simulink model "XY_1_pen_sim"  (R2024b)
settings: Solver=ode4  StartTime=0.0  StopTime=T_run  FixedStep=Ts_plant  RelTol=1e-3
StopFcn:
  | XY_stop
values from neighbouring files (symbols this model uses):
  alpha_s = 0    [XY_setup.m]
  anim_Ts = 0.2    [XY_setup.m]
  animate = 1    [XY_1_pen_sim_run.m]    (also in XY_compare.m = 0; XY_run_all.m; XY_setup.m)
  B_eff = 0.30    (= 0.3)    [XY_setup.m]
  b_trk = 0.28    [XY_setup.m]
  d_reach = 0.03    [XY_setup.m]
  db_v = 47    [XY_setup.m]
  db_w = 20    [XY_setup.m]
  dist_p = [slip_k; wob_amp; wob_f]    [XY_setup.m]
  dyn_p = [m_r; l_trk; b_trk; mu_l; mu_t; N_mag; g_acc]    [XY_setup.m]
  F_max = 200    [XY_setup.m]
  imu_drift = deg2rad(0.02)    [XY_setup.m]
  imu_sigma = deg2rad(0.3)    [XY_setup.m]
  imu_Ts = 0.01    [XY_setup.m]
  K_c = 0    [XY_setup.m]
  K_ci = 0    [XY_setup.m]
  K_dist = 1.0    (= 1)    [XY_setup.m]
  K_ptheta = 1.4    [XY_setup.m]
  k_pwm = v_full/(400 - pwm_dz)    (= 0.000540540540541)    [XY_setup.m]
  K_px = 0.3    [XY_setup.m]
  K_py = 5.0    (= 5)    [XY_setup.m]
  K_yaw = 2.0    (= 2)    [XY_setup.m]
  Ki_v = 15000    [XY_setup.m]
  Ki_w = 15000    [XY_setup.m]
  Kp_v = 1500    [XY_setup.m]
  Kp_w = 1500    [XY_setup.m]
  L_r = sqrt((l_trk^2 + b_trk^2)/12)    [XY_setup.m]
  line_post = 0.04    [XY_setup.m]
  line_pre = 0.06    [XY_setup.m]
  pen_A = [-0.70; 0.30]    [XY_setup.m]
  pen_B = [ 0.50; 0.30]    [XY_setup.m]
  pen_d = r_pen0 - r_tag    [XY_setup.m]
  psi0 = pi/2    (= 1.57079632679)    [XY_setup.m]
  pwm_dz = 30    [XY_setup.m]
  q0 = [-0.85; 0.10; pi/2]    [XY_setup.m]
  q0c = [q0(1:2) - [cos(q0(3)) -sin(q0(3)); sin(q0(3)) cos(q0(3))] * r_tag; q0(3)]    [XY_setup.m]
  r_tag = [-0.080;  0.060]    [XY_setup.m]
  stage_acc = 500    [XY_setup.m]
  stage_c = stage_travel/2    (= 50.8)    [XY_setup.m]
  stage_cmd_Ts = 0.04    [XY_setup.m]
  stage_delay = 0.01    [XY_setup.m]
  stage_Fv_F = [32 32 29 26.5 25 22  20 17.5 14  9]    [XY_setup.m]
  stage_Fv_v = [0  2  7  13  20  32  45  60  80  104]    [XY_setup.m]
  stage_travel = 101.6    [XY_setup.m]
  stage_Ts = 0.05    [XY_setup.m]
  stage_vcmd = 0.8*stage_vmax    (= 83.2)    [XY_setup.m]
  stage_vmax = 104    [XY_setup.m]
  stg_p = [m_sx; m_sy; c_s; Kp_s; Kd_s; Ki_s; g_acc]    [XY_compare.m]    (also in XY_setup.m)
  tau_pred = 0    [XY_setup.m]
  th_tol = deg2rad(1)    [XY_setup.m]
  trk_A = -eye(2)/tau_trk    [XY_setup.m]
  trk_B = eye(2)/tau_trk    [XY_setup.m]
  trk_C = eye(2)    [XY_setup.m]
  trk_D = zeros(2)    [XY_setup.m]
  Ts_ctrl = 0.01    [XY_setup.m]
  v_full = 0.20    (= 0.2)    [XY_setup.m]
  v_max = 0.20    (= 0.2)    [XY_setup.m]
  v_ref = 0.03    [XY_setup.m]
  w_full = 2*k_pwm*(400 - db_w)/B_eff    (= 1.36936936937)    [XY_setup.m]
  w_max = deg2rad(45)    [XY_setup.m]
  x = c(1) + s(1)/2*[-1 1 1 -1 -1 1 1 -1]    [XY_animate.m]
  x_s0 = [stage_c; stage_c; 0; 0; 0; 0] .* [1e-3; 1e-3; 1; 1; 1; 1]    [XY_setup.m]
  x_t0 = [stage_c; stage_c; 0; 0]    [XY_setup.m]
  y = c(2) + s(2)/2*[-1 -1 1 1 -1 -1 1 1]    [XY_animate.m]    (also in build_xy_models.m = q(2))
  zk_delay = 0.05    [XY_setup.m]
  zk_sigma = 0.0010    (= 0.001)    [XY_setup.m]
  zk_Ts = 0.05    [XY_setup.m]
  zk_xsign = -1    [XY_setup.m]
  zk_ywall = 0.02    [XY_setup.m]
undefined symbols (not defined in the file or in its folder): orientation, point, quaternion, twist
libraries: ros2lib x20, simulink x4, slpidlib x2
(part 1 of 2)
settings Model: PacingRate=4  Creator=admin  LastModifiedBy=admin
settings DataIOCC: ReturnWorkspaceOutputs=off

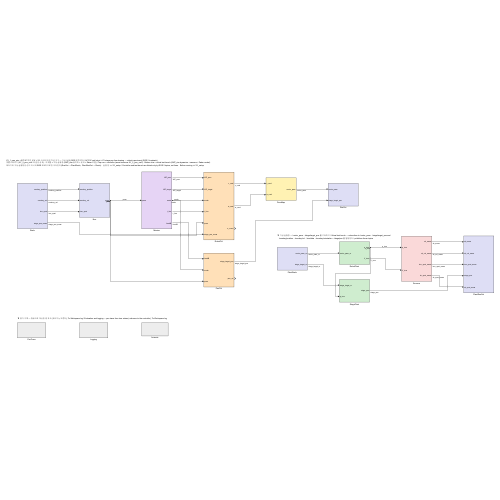
[thumbnail: Simulink's stored preview of the top-level diagram]
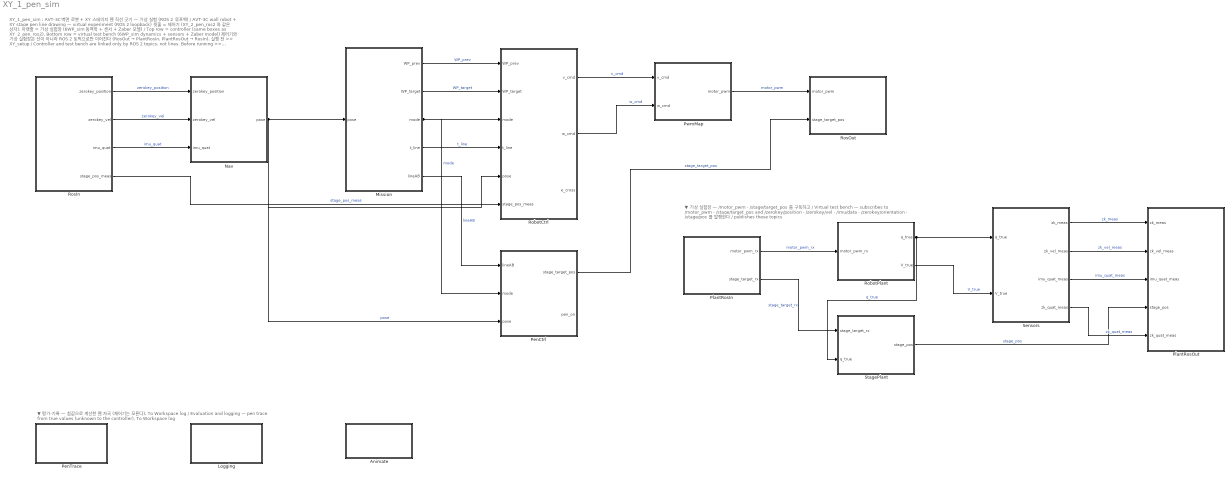
== system XY_1_pen_sim ==
  note: XY_1_pen_sim : AVT-3C 벽면 로봇 + XY 스테이지 펜 직선 긋기 — 가상 실험 (ROS 2 루프백) / AVT-3C wall robot + XY stage pen line drawing — virtual experiment (ROS 2 loopback)
      | 윗줄 = 제어기 (XY_2_pen_ros2 와 같은 상자).  아랫줄 = 가상 실험장 (6WP_sim 동역학 + 센서 + Zaber 모델) / Top row = controller (same boxes as XY_2_pen_ros2).  Bottom row = virtual test bench (6WP_sim dynamics + sensors + Zaber model)
      | 제어기와 가상 실험장은 선이 아니라 ROS 2 토픽으로만 이어진다 (RosOut → PlantRosIn,  PlantRosOut → RosIn).   실행 전 >> XY_setup / Controller and test bench are linked only by ROS 2 topics, not lines.   Before running >> XY_setup
  note: ▼ 가상 실험장 — /motor_pwm · /stage/target_pos 를 구독하고 / Virtual test bench — subscribes to /motor_pwm · /stage/target_pos and
      |    /zerokey/position · /zerokey/vel · /imu/data · /zerokey/orientation · /stage/pos 를 발행한다 / publishes these topics
  note: ▼ 평가·기록 — 참값으로 계산한 펜 자국 (제어기는 모른다), To Workspace log / Evaluation and logging — pen trace from true values (unknown to the controller), To Workspace log
  Animate : Subsystem
  Logging : Subsystem
  Mission : Subsystem
  Nav : Subsystem
  PenCtrl : Subsystem
  PenTrace : Subsystem
  PlantRosIn : Subsystem
  PlantRosOut : Subsystem
  PwmMap : Subsystem
  RobotCtrl : Subsystem
  RobotPlant : Subsystem
  RosIn : Subsystem
  RosOut : Subsystem
  Sensors : Subsystem
  StagePlant : Subsystem
  wires:
  Nav/1(pose) -> Mission/1(pose), PenCtrl/3(pose), RobotCtrl/5(pose)  "pose"
  RosIn/1(zerokey_position) -> Nav/1(zerokey_position)  "zerokey_position"
  RosIn/2(zerokey_vel) -> Nav/2(zerokey_vel)  "zerokey_vel"
  RosIn/3(imu_quat) -> Nav/3(imu_quat)  "imu_quat"
  Mission/5(lineAB) -> PenCtrl/1(lineAB)  "lineAB"
  Mission/3(mode) -> PenCtrl/2(mode), RobotCtrl/3(mode)  "mode"
  Sensors/1(zk_meas) -> PlantRosOut/1(zk_meas)  "zk_meas"
  Sensors/2(zk_vel_meas) -> PlantRosOut/2(zk_vel_meas)  "zk_vel_meas"
  Sensors/3(imu_quat_meas) -> PlantRosOut/3(imu_quat_meas)  "imu_quat_meas"
  StagePlant/1(stage_pos) -> PlantRosOut/4(stage_pos)  "stage_pos"
  Sensors/4(zk_quat_meas) -> PlantRosOut/5(zk_quat_meas)  "zk_quat_meas"
  RobotCtrl/1(v_cmd) -> PwmMap/1(v_cmd)  "v_cmd"
  RobotCtrl/2(w_cmd) -> PwmMap/2(w_cmd)  "w_cmd"
  Mission/1(WP_prev) -> RobotCtrl/1(WP_prev)  "WP_prev"
  Mission/2(WP_target) -> RobotCtrl/2(WP_target)  "WP_target"
  Mission/4(t_line) -> RobotCtrl/4(t_line)  "t_line"
  RosIn/4(stage_pos_meas) -> RobotCtrl/6(stage_pos_meas)  "stage_pos_meas"
  PlantRosIn/1(motor_pwm_rx) -> RobotPlant/1(motor_pwm_rx)  "motor_pwm_rx"
  PwmMap/1(motor_pwm) -> RosOut/1(motor_pwm)  "motor_pwm"
  PenCtrl/1(stage_target_pos) -> RosOut/2(stage_target_pos)  "stage_target_pos"
  RobotPlant/1(q_true) -> Sensors/1(q_true), StagePlant/2(q_true)  "q_true"
  RobotPlant/2(V_true) -> Sensors/2(V_true)  "V_true"
  PlantRosIn/2(stage_target_rx) -> StagePlant/1(stage_target_rx)  "stage_target_rx"

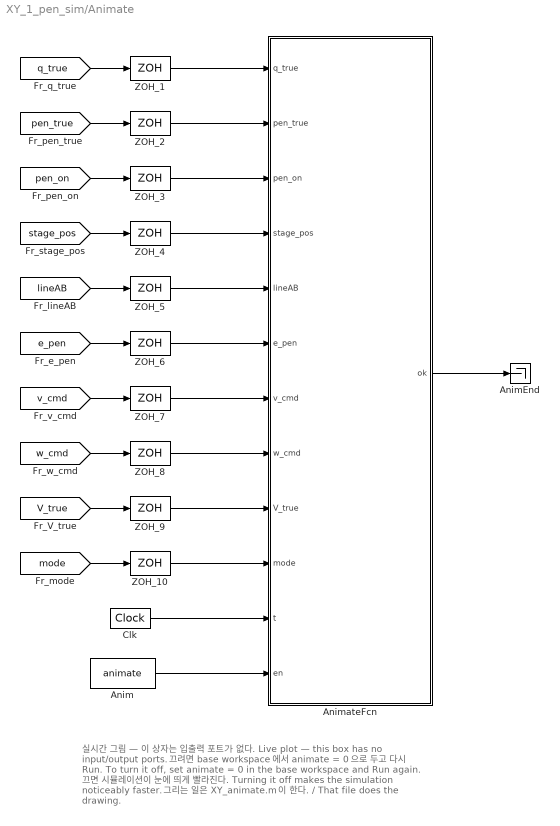
== system XY_1_pen_sim/Animate ==
  note: 실시간 그림 — 이 상자는 입출력 포트가 없다.
      | Live plot — this box has no input/output ports.
      | 끄려면 base workspace 에서  animate = 0  으로 두고 다시 Run.
      | To turn it off, set  animate = 0  in the base workspace and Run again.
      | 끄면 시뮬레이션이 눈에 띄게 빨라진다.
      | Turning it off makes the simulation noticeably faster.
      | 그리는 일은 XY_animate.m 이 한다. / That file does the drawing.
  Anim : Constant  Value=animate
  AnimEnd : Terminator
  AnimateFcn : MATLAB Function  TreatAsAtomicUnit=on
  Clk : DigitalClock  SampleTime=anim_Ts
  ZOH_{1..10} (10 alike) : ZeroOrderHold  SampleTime=anim_Ts
  wires:
  Clk/1 -> AnimateFcn/11(t)
  Anim/1 -> AnimateFcn/12(en)
  AnimateFcn/1(ok) -> AnimEnd/1
  [q_true] -> ZOH_1/1
  ZOH_1/1 -> AnimateFcn/1(q_true)
  [pen_true] -> ZOH_2/1
  ZOH_2/1 -> AnimateFcn/2(pen_true)
  [pen_on] -> ZOH_3/1
  ZOH_3/1 -> AnimateFcn/3(pen_on)
  [stage_pos] -> ZOH_4/1
  ZOH_4/1 -> AnimateFcn/4(stage_pos)
  [lineAB] -> ZOH_5/1
  ZOH_5/1 -> AnimateFcn/5(lineAB)
  [e_pen] -> ZOH_6/1
  ZOH_6/1 -> AnimateFcn/6(e_pen)
  [v_cmd] -> ZOH_7/1
  ZOH_7/1 -> AnimateFcn/7(v_cmd)
  [w_cmd] -> ZOH_8/1
  ZOH_8/1 -> AnimateFcn/8(w_cmd)
  [V_true] -> ZOH_9/1
  ZOH_9/1 -> AnimateFcn/9(V_true)
  [mode] -> ZOH_10/1
  ZOH_10/1 -> AnimateFcn/10(mode)

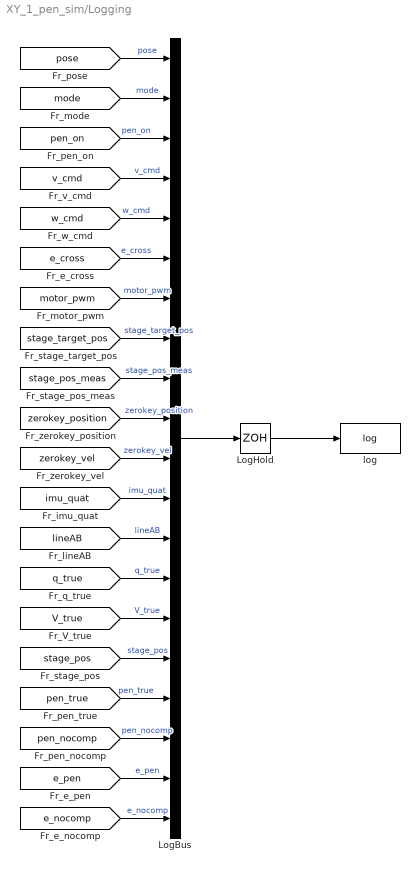
== system XY_1_pen_sim/Logging ==
  LogBus : BusCreator  Inputs=20
  LogHold : ZeroOrderHold  Description=이산: 기록 주기 (제어기 주기와 같다) / Discrete: logging period (same as the controller period)  SampleTime=Ts_ctrl
  log : ToWorkspace  VariableName=log  SaveFormat=Timeseries  SampleTime=Ts_ctrl
  wires:
  [pose] -> LogBus/1  "pose"
  [mode] -> LogBus/2  "mode"
  [pen_on] -> LogBus/3  "pen_on"
  [v_cmd] -> LogBus/4  "v_cmd"
  [w_cmd] -> LogBus/5  "w_cmd"
  [e_cross] -> LogBus/6  "e_cross"
  [motor_pwm] -> LogBus/7  "motor_pwm"
  [stage_target_pos] -> LogBus/8  "stage_target_pos"
  [stage_pos_meas] -> LogBus/9  "stage_pos_meas"
  [zerokey_position] -> LogBus/10  "zerokey_position"
  [zerokey_vel] -> LogBus/11  "zerokey_vel"
  [imu_quat] -> LogBus/12  "imu_quat"
  [lineAB] -> LogBus/13  "lineAB"
  [q_true] -> LogBus/14  "q_true"
  [V_true] -> LogBus/15  "V_true"
  [stage_pos] -> LogBus/16  "stage_pos"
  [pen_true] -> LogBus/17  "pen_true"
  [pen_nocomp] -> LogBus/18  "pen_nocomp"
  [e_pen] -> LogBus/19  "e_pen"
  [e_nocomp] -> LogBus/20  "e_nocomp"
  LogBus/1 -> LogHold/1
  LogHold/1 -> log/1

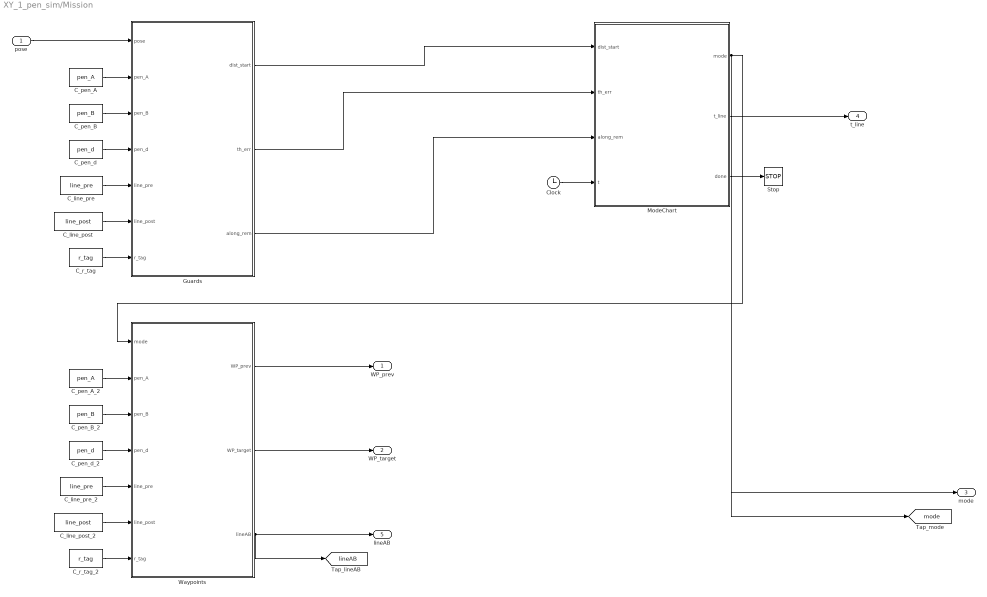
== system XY_1_pen_sim/Mission ==
  pose : Inport
  C_line_post : Constant  Value=line_post
  C_line_post_2 : Constant  Value=line_post
  C_line_pre : Constant  Value=line_pre
  C_line_pre_2 : Constant  Value=line_pre
  C_pen_A : Constant  Value=pen_A
  C_pen_A_2 : Constant  Value=pen_A
  C_pen_B : Constant  Value=pen_B
  C_pen_B_2 : Constant  Value=pen_B
  C_pen_d : Constant  Value=pen_d
  C_pen_d_2 : Constant  Value=pen_d
  C_r_tag : Constant  Value=r_tag
  C_r_tag_2 : Constant  Value=r_tag
  Clock : Clock
  Guards : MATLAB Function  TreatAsAtomicUnit=on
  ModeChart : Stateflow chart  Description=이산: 모드는 사건 상태 (6WP_sim Chart 와 같은 역할). 전이: 거리 < d_reach, 1 s 뒤 각 오차 < th_tol, 남은 거리 < d_reach, 정지 2 s / Discrete: the mode is an event state (same role as the 6WP_sim Chart). Transitions: distance < d_reach, angle error < th_tol after 1 s, remaining distance < d_reach, stop 2 s  TreatAsAtomicUnit=on
  Stop : Stop
  Waypoints : MATLAB Function  TreatAsAtomicUnit=on
  WP_prev : Outport
  WP_target : Outport  Port=2
  mode : Outport  Port=3
  t_line : Outport  Port=4
  lineAB : Outport  Port=5
  tag scope: lineAB=global, mode=global
  wires:
  pose/1 -> Guards/1(pose)
  C_pen_A/1 -> Guards/2(pen_A)
  C_pen_B/1 -> Guards/3(pen_B)
  C_pen_d/1 -> Guards/4(pen_d)
  C_line_pre/1 -> Guards/5(line_pre)
  C_line_post/1 -> Guards/6(line_post)
  C_r_tag/1 -> Guards/7(r_tag)
  Clock/1 -> ModeChart/4(t)
  ModeChart/2(t_line) -> t_line/1
  ModeChart/3(done) -> Stop/1
  C_pen_A_2/1 -> Waypoints/2(pen_A)
  C_pen_B_2/1 -> Waypoints/3(pen_B)
  C_pen_d_2/1 -> Waypoints/4(pen_d)
  C_line_pre_2/1 -> Waypoints/5(line_pre)
  C_line_post_2/1 -> Waypoints/6(line_post)
  C_r_tag_2/1 -> Waypoints/7(r_tag)
  Waypoints/1(WP_prev) -> WP_prev/1
  Waypoints/2(WP_target) -> WP_target/1
  Waypoints/3(lineAB) -> lineAB/1, [lineAB]
  Guards/3(along_rem) -> ModeChart/3(along_rem)
  Guards/1(dist_start) -> ModeChart/1(dist_start)
  ModeChart/1(mode) -> Waypoints/1(mode), mode/1, [mode]
  Guards/2(th_err) -> ModeChart/2(th_err)

== system XY_1_pen_sim/Nav ==
  zerokey_position : Inport
  zerokey_vel : Inport  Port=2
  imu_quat : Inport  Port=3
  C_psi0 : Constant  Value=psi0
  C_tau_pred : Constant  Value=tau_pred
  C_zk_xsign : Constant  Value=zk_xsign
  NavFcn : MATLAB Function  Description=이산: persistent (첫 요각 기억) — 구독 주기와 같다 / Discrete: persistent (stores the first yaw) — same as the subscription period  TreatAsAtomicUnit=on
  pose : Outport
  tag scope: pose=global
  wires:
  zerokey_position/1 -> NavFcn/1(zerokey_position)
  zerokey_vel/1 -> NavFcn/2(zerokey_vel)
  imu_quat/1 -> NavFcn/3(imu_quat)
  C_psi0/1 -> NavFcn/4(psi0)
  C_tau_pred/1 -> NavFcn/5(tau_pred)
  C_zk_xsign/1 -> NavFcn/6(zk_xsign)
  NavFcn/1(pose) -> pose/1, [pose]

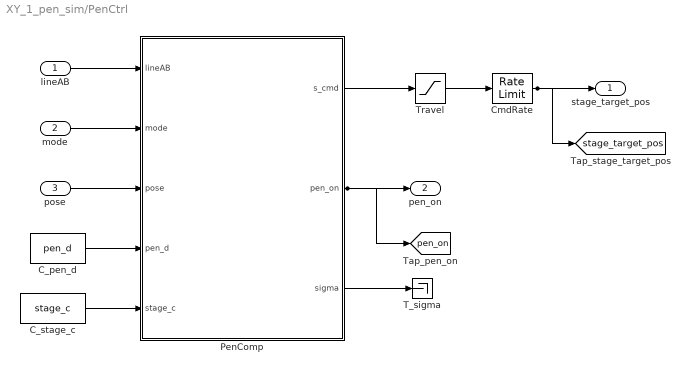
== system XY_1_pen_sim/PenCtrl ==
  lineAB : Inport
  mode : Inport  Port=2
  pose : Inport  Port=3
  C_pen_d : Constant  Value=pen_d
  C_stage_c : Constant  Value=stage_c
  CmdRate : RateLimiter  RisingSlewLimit=stage_vcmd  FallingSlewLimit=-stage_vcmd  SampleTimeMode=inherited  InitialCondition=stage_c
  PenComp : MATLAB Function  TreatAsAtomicUnit=on
  T_sigma : Terminator
  Travel : Saturate  UpperLimit=stage_travel  LowerLimit=0
  stage_target_pos : Outport
  pen_on : Outport  Port=2
  tag scope: pen_on=global, stage_target_pos=global
  wires:
  pose/1 -> PenComp/3(pose)
  lineAB/1 -> PenComp/1(lineAB)
  PenComp/1(s_cmd) -> Travel/1
  C_stage_c/1 -> PenComp/5(stage_c)
  C_pen_d/1 -> PenComp/4(pen_d)
  mode/1 -> PenComp/2(mode)
  PenComp/2(pen_on) -> pen_on/1, [pen_on]
  PenComp/3(sigma) -> T_sigma/1
  Travel/1 -> CmdRate/1
  CmdRate/1 -> stage_target_pos/1, [stage_target_pos]

== system XY_1_pen_sim/PenTrace ==
  C_pen_d : Constant  Value=pen_d
  C_stage_c : Constant  Value=stage_c
  PenTraceFcn : MATLAB Function  TreatAsAtomicUnit=on
  tag scope: e_nocomp=global, e_pen=global, pen_nocomp=global, pen_true=global
  wires:
  [q_true] -> PenTraceFcn/1(q_true)
  [stage_pos] -> PenTraceFcn/2(stage_pos)
  [lineAB] -> PenTraceFcn/3(lineAB)
  C_pen_d/1 -> PenTraceFcn/4(pen_d)
  C_stage_c/1 -> PenTraceFcn/5(stage_c)
  PenTraceFcn/1(pen_true) -> [pen_true]
  PenTraceFcn/2(pen_nocomp) -> [pen_nocomp]
  PenTraceFcn/3(e_pen) -> [e_pen]
  PenTraceFcn/4(e_nocomp) -> [e_nocomp]

== system XY_1_pen_sim/PlantRosIn ==
  IsNew_SubPwm : Terminator
  IsNew_SubStg : Terminator
  Mux_SubPwm : Mux  Inputs=2
  Mux_SubStg : Mux  Inputs=2
  Sel_SubPwm : BusSelector  OutputSignals=x,y
  Sel_SubStg : BusSelector  OutputSignals=x,y
  SubPwm : ros2lib/Subscribe  Description=이산: ROS Subscribe 는 구독 주기로만 돈다 / Discrete: ROS Subscribe runs only at the subscription period  topicSource=Specify your own  topic=/motor_pwm  messageType=geometry_msgs/Point  sampleTime=Ts_ctrl  QOSHistory=Keep last  QOSDepth=1  QOSReliability=Reliable  QOSDurability=Volatile  QOSDeadline=Inf  QOSLifespan=Inf  QOSLiveliness=Automatic  QOSLeaseDuration=Inf  QOSAvoidROSNamespaceConventions=off
  SubStg : ros2lib/Subscribe  Description=이산: ROS Subscribe 는 구독 주기로만 돈다 / Discrete: ROS Subscribe runs only at the subscription period  topicSource=Specify your own  topic=/stage/target_pos  messageType=geometry_msgs/Point  sampleTime=Ts_ctrl  QOSHistory=Keep last  QOSDepth=1  QOSReliability=Reliable  QOSDurability=Volatile  QOSDeadline=Inf  QOSLifespan=Inf  QOSLiveliness=Automatic  QOSLeaseDuration=Inf  QOSAvoidROSNamespaceConventions=off
  motor_pwm_rx : Outport
  stage_target_rx : Outport  Port=2
  wires:
  SubPwm/2 -> Sel_SubPwm/1
  SubPwm/1 -> IsNew_SubPwm/1
  Sel_SubPwm/1 -> Mux_SubPwm/1  "<x>"
  Sel_SubPwm/2 -> Mux_SubPwm/2  "<y>"
  Mux_SubPwm/1 -> motor_pwm_rx/1
  SubStg/2 -> Sel_SubStg/1
  SubStg/1 -> IsNew_SubStg/1
  Sel_SubStg/1 -> Mux_SubStg/1  "<x>"
  Sel_SubStg/2 -> Mux_SubStg/2  "<y>"
  Mux_SubStg/1 -> stage_target_rx/1

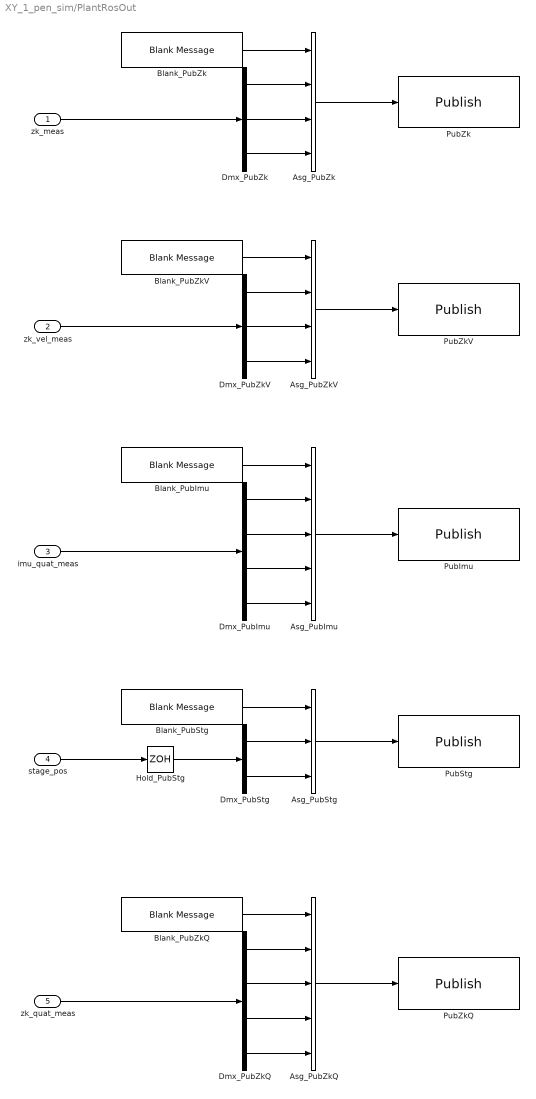
== system XY_1_pen_sim/PlantRosOut ==
  zk_meas : Inport
  zk_vel_meas : Inport  Port=2
  imu_quat_meas : Inport  Port=3
  stage_pos : Inport  Port=4
  zk_quat_meas : Inport  Port=5
  Asg_PubImu : BusAssignment  AssignedSignals=orientation.w,orientation.x,orientation.y,orientation.z
  Asg_PubStg : BusAssignment  AssignedSignals=point.x,point.y
  Asg_PubZk : BusAssignment  AssignedSignals=point.x,point.y,point.z
  Asg_PubZkQ : BusAssignment  AssignedSignals=quaternion.w,quaternion.x,quaternion.y,quaternion.z
  Asg_PubZkV : BusAssignment  AssignedSignals=twist.linear.x,twist.linear.y,twist.linear.z
  Blank_PubImu : ros2lib/Blank Message  messageClass=Message  entityType=sensor_msgs/Imu  messageType=sensor_msgs/Imu  SampleTime=inf
  Blank_PubStg : ros2lib/Blank Message  messageClass=Message  entityType=geometry_msgs/PointStamped  messageType=geometry_msgs/PointStamped  SampleTime=inf
  Blank_PubZk : ros2lib/Blank Message  messageClass=Message  entityType=geometry_msgs/PointStamped  messageType=geometry_msgs/PointStamped  SampleTime=inf
  Blank_PubZkQ : ros2lib/Blank Message  messageClass=Message  entityType=geometry_msgs/QuaternionStamped  messageType=geometry_msgs/QuaternionStamped  SampleTime=inf
  Blank_PubZkV : ros2lib/Blank Message  messageClass=Message  entityType=geometry_msgs/TwistStamped  messageType=geometry_msgs/TwistStamped  SampleTime=inf
  Dmx_PubImu : Demux
  Dmx_PubStg : Demux  Outputs=2
  Dmx_PubZk : Demux  Outputs=3
  Dmx_PubZkQ : Demux
  Dmx_PubZkV : Demux  Outputs=3
  Hold_PubStg : ZeroOrderHold  Description=이산: 발행 주기 / Discrete: publish period  SampleTime=stage_Ts
  PubImu : ros2lib/Publish  topicSource=Specify your own  topic=/imu/data  messageType=sensor_msgs/Imu  QOSHistory=Keep last  QOSDepth=1  QOSReliability=Reliable  QOSDurability=Volatile  QOSDeadline=Inf  QOSLifespan=Inf  QOSLiveliness=Automatic  QOSLeaseDuration=Inf  QOSAvoidROSNamespaceConventions=off
  PubStg : ros2lib/Publish  topicSource=Specify your own  topic=/stage/pos  messageType=geometry_msgs/PointStamped  QOSHistory=Keep last  QOSDepth=1  QOSReliability=Reliable  QOSDurability=Volatile  QOSDeadline=Inf  QOSLifespan=Inf  QOSLiveliness=Automatic  QOSLeaseDuration=Inf  QOSAvoidROSNamespaceConventions=off
  PubZk : ros2lib/Publish  topicSource=Specify your own  topic=/zerokey/position  messageType=geometry_msgs/PointStamped  QOSHistory=Keep last  QOSDepth=1  QOSReliability=Reliable  QOSDurability=Volatile  QOSDeadline=Inf  QOSLifespan=Inf  QOSLiveliness=Automatic  QOSLeaseDuration=Inf  QOSAvoidROSNamespaceConventions=off
  PubZkQ : ros2lib/Publish  topicSource=Specify your own  topic=/zerokey/orientation  messageType=geometry_msgs/QuaternionStamped  QOSHistory=Keep last  QOSDepth=1  QOSReliability=Reliable  QOSDurability=Volatile  QOSDeadline=Inf  QOSLifespan=Inf  QOSLiveliness=Automatic  QOSLeaseDuration=Inf  QOSAvoidROSNamespaceConventions=off
  PubZkV : ros2lib/Publish  topicSource=Specify your own  topic=/zerokey/vel  messageType=geometry_msgs/TwistStamped  QOSHistory=Keep last  QOSDepth=1  QOSReliability=Reliable  QOSDurability=Volatile  QOSDeadline=Inf  QOSLifespan=Inf  QOSLiveliness=Automatic  QOSLeaseDuration=Inf  QOSAvoidROSNamespaceConventions=off
  wires:
  Blank_PubZk/1 -> Asg_PubZk/1
  Dmx_PubZk/1 -> Asg_PubZk/2
  Dmx_PubZk/2 -> Asg_PubZk/3
  Dmx_PubZk/3 -> Asg_PubZk/4
  zk_meas/1 -> Dmx_PubZk/1
  Asg_PubZk/1 -> PubZk/1
  Blank_PubZkV/1 -> Asg_PubZkV/1
  Dmx_PubZkV/1 -> Asg_PubZkV/2
  Dmx_PubZkV/2 -> Asg_PubZkV/3
  Dmx_PubZkV/3 -> Asg_PubZkV/4
  zk_vel_meas/1 -> Dmx_PubZkV/1
  Asg_PubZkV/1 -> PubZkV/1
  Blank_PubImu/1 -> Asg_PubImu/1
  Dmx_PubImu/1 -> Asg_PubImu/2
  Dmx_PubImu/2 -> Asg_PubImu/3
  Dmx_PubImu/3 -> Asg_PubImu/4
  Dmx_PubImu/4 -> Asg_PubImu/5
  imu_quat_meas/1 -> Dmx_PubImu/1
  Asg_PubImu/1 -> PubImu/1
  Blank_PubStg/1 -> Asg_PubStg/1
  Dmx_PubStg/1 -> Asg_PubStg/2
  Dmx_PubStg/2 -> Asg_PubStg/3
  Hold_PubStg/1 -> Dmx_PubStg/1
  stage_pos/1 -> Hold_PubStg/1
  Asg_PubStg/1 -> PubStg/1
  Blank_PubZkQ/1 -> Asg_PubZkQ/1
  Dmx_PubZkQ/1 -> Asg_PubZkQ/2
  Dmx_PubZkQ/2 -> Asg_PubZkQ/3
  Dmx_PubZkQ/3 -> Asg_PubZkQ/4
  Dmx_PubZkQ/4 -> Asg_PubZkQ/5
  zk_quat_meas/1 -> Dmx_PubZkQ/1
  Asg_PubZkQ/1 -> PubZkQ/1

== system XY_1_pen_sim/PwmMap ==
  v_cmd : Inport
  w_cmd : Inport  Port=2
  C_db_v : Constant  Value=db_v
  C_db_w : Constant  Value=db_w
  C_v_full : Constant  Value=v_full
  C_w_full : Constant  Value=w_full
  calc_pwm : MATLAB Function  TreatAsAtomicUnit=on
  motor_pwm : Outport
  tag scope: motor_pwm=global
  wires:
  v_cmd/1 -> calc_pwm/1(v_cmd)
  w_cmd/1 -> calc_pwm/2(w_cmd)
  C_v_full/1 -> calc_pwm/3(v_full)
  C_w_full/1 -> calc_pwm/4(w_full)
  C_db_v/1 -> calc_pwm/5(db_v)
  C_db_w/1 -> calc_pwm/6(db_w)
  calc_pwm/1(motor_pwm) -> motor_pwm/1, [motor_pwm]

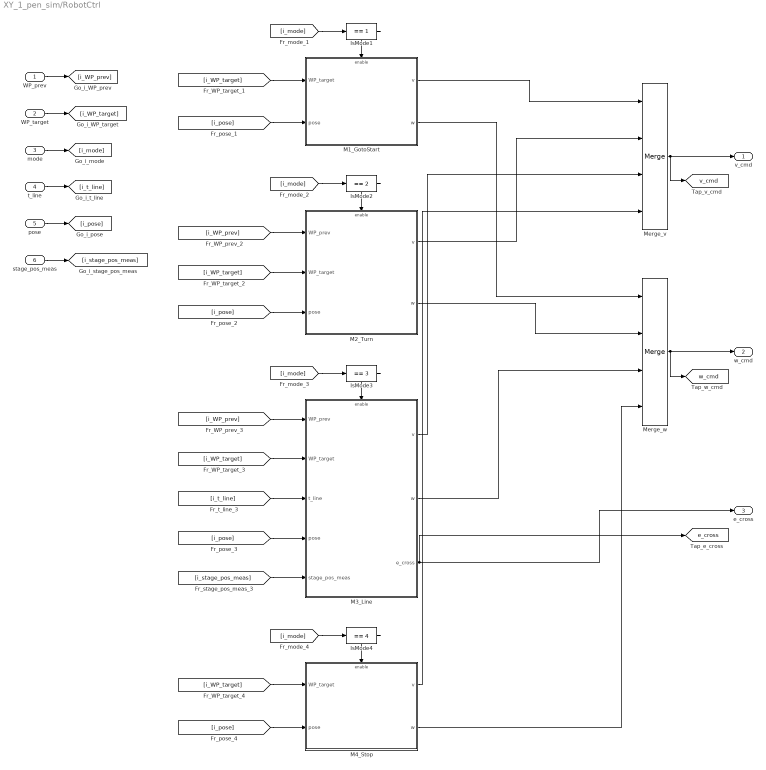
== system XY_1_pen_sim/RobotCtrl ==
  WP_prev : Inport
  WP_target : Inport  Port=2
  mode : Inport  Port=3
  t_line : Inport  Port=4
  pose : Inport  Port=5
  stage_pos_meas : Inport  Port=6
  IsMode1 : simulink/Logic and Bit Operations/Compare To Constant  relop===  const=1  OutDataTypeStr=boolean
  IsMode2 : simulink/Logic and Bit Operations/Compare To Constant  relop===  const=2  OutDataTypeStr=boolean
  IsMode3 : simulink/Logic and Bit Operations/Compare To Constant  relop===  const=3  OutDataTypeStr=boolean
  IsMode4 : simulink/Logic and Bit Operations/Compare To Constant  relop===  const=4  OutDataTypeStr=boolean
  M1_GotoStart : Subsystem
  M2_Turn : Subsystem
  M3_Line : Subsystem
  M4_Stop : Subsystem
  Merge_v : Merge  Inputs=4
  Merge_w : Merge  Inputs=4
  v_cmd : Outport
  w_cmd : Outport  Port=2
  e_cross : Outport  Port=3
  tag scope: e_cross=global, v_cmd=global, w_cmd=global
  wires:
  WP_prev/1 -> [i_WP_prev]
  WP_target/1 -> [i_WP_target]
  mode/1 -> [i_mode]
  t_line/1 -> [i_t_line]
  pose/1 -> [i_pose]
  stage_pos_meas/1 -> [i_stage_pos_meas]
  [i_WP_target] -> M1_GotoStart/1(WP_target)
  [i_pose] -> M1_GotoStart/2(pose)
  [i_mode] -> IsMode1/1
  IsMode1/1 -> M1_GotoStart/Enable
  [i_WP_prev] -> M2_Turn/1(WP_prev)
  [i_WP_target] -> M2_Turn/2(WP_target)
  [i_pose] -> M2_Turn/3(pose)
  [i_mode] -> IsMode2/1
  IsMode2/1 -> M2_Turn/Enable
  [i_WP_prev] -> M3_Line/1(WP_prev)
  [i_WP_target] -> M3_Line/2(WP_target)
  [i_t_line] -> M3_Line/3(t_line)
  [i_pose] -> M3_Line/4(pose)
  [i_stage_pos_meas] -> M3_Line/5(stage_pos_meas)
  [i_mode] -> IsMode3/1
  IsMode3/1 -> M3_Line/Enable
  [i_WP_target] -> M4_Stop/1(WP_target)
  [i_pose] -> M4_Stop/2(pose)
  [i_mode] -> IsMode4/1
  IsMode4/1 -> M4_Stop/Enable
  Merge_v/1 -> v_cmd/1, [v_cmd]
  Merge_w/1 -> w_cmd/1, [w_cmd]
  M3_Line/3(e_cross) -> e_cross/1, [e_cross]
  M1_GotoStart/1(v) -> Merge_v/1
  M2_Turn/1(v) -> Merge_v/2
  M3_Line/1(v) -> Merge_v/3
  M4_Stop/1(v) -> Merge_v/4
  M1_GotoStart/2(w) -> Merge_w/1
  M2_Turn/2(w) -> Merge_w/2
  M3_Line/2(w) -> Merge_w/3
  M4_Stop/2(w) -> Merge_w/4

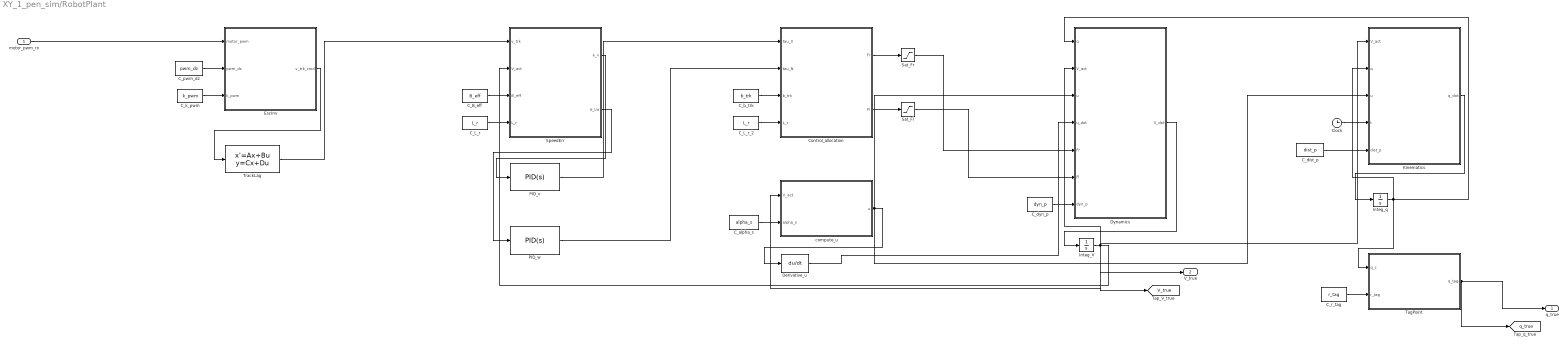
== system XY_1_pen_sim/RobotPlant ==
  motor_pwm_rx : Inport
  C_B_eff : Constant  Value=B_eff
  C_L_r : Constant  Value=L_r
  C_L_r_2 : Constant  Value=L_r
  C_alpha_s : Constant  Value=alpha_s
  C_b_trk : Constant  Value=b_trk
  C_dist_p : Constant  Value=dist_p
  C_dyn_p : Constant  Value=dyn_p
  C_k_pwm : Constant  Value=k_pwm
  C_pwm_dz : Constant  Value=pwm_dz
  C_r_tag : Constant  Value=r_tag
  Clock : Clock
  Control_allocation : MATLAB Function  TreatAsAtomicUnit=on
  Derivative_u : Derivative
  Dynamics : MATLAB Function  TreatAsAtomicUnit=on
  EscInv : MATLAB Function  TreatAsAtomicUnit=on
  Integ_V : Integrator  InitialCondition=[0;0]
  Integ_q : Integrator  InitialCondition=q0c
  Kinematics : MATLAB Function  TreatAsAtomicUnit=on
  PID_v : slpidlib/PID Controller  Controller=PID  Form=Parallel  TimeDomain=Continuous-time  UseExternalTs=off  SampleTime=-1  IntegratorMethod=Forward Euler  FilterMethod=Forward Euler  ControllerParametersSource=internal  P=Kp_v  I=Ki_v  UseKiTs=off  D=0  UseExternalDerivativeSource=off  N=100  UseFilter=on  TunerSelectOption=Transfer Function Based (PID Tuner App)  InitialConditionSource=internal  InitialConditionForIntegrator=0  InitialConditionForFilter=0  DifferentiatorICPrevScaledInput=0  ExternalReset=none  TrackingMode=off  Kt=1  LimitOutput=off  SatLimitsSource=internal  UpperSaturationLimit=inf  LowerSaturationLimit=-inf  LinearizeAsGain=on  AntiWindupMode=none  Kb=1  LimitIntegrator=off  UpperIntegratorSaturationLimit=inf  LowerIntegratorSaturationLimit=-inf  POutMin=[]  POutMax=[]  IOutMin=[]  IOutMax=[]  DOutMin=[]  DOutMax=[]  NOutMin=[]  NOutMax=[]  SumOutMin=[]  SumOutMax=[]  SaturationOutMin=[]  SaturationOutMax=[]  PParamMin=[]  PParamMax=[]  IParamMin=[]  IParamMax=[]  DParamMin=[]  DParamMax=[]  NParamMin=[]  NParamMax=[]  KbParamMin=[]  KbParamMax=[]  KtParamMin=[]  KtParamMax=[]  KbOutMin=[]  KbOutMax=[]  KtOutMin=[]  KtOutMax=[]  IntegratorOutMin=[]  IntegratorOutMax=[]  FilterOutMin=[]  FilterOutMax=[]  SumI1OutMin=[]  SumI1OutMax=[]  SumI2OutMin=[]  SumI2OutMax=[]  SumI3OutMin=[]  SumI3OutMax=[]  SumI4OutMin=[]  SumI4OutMax=[]  SumDOutMin=[]  SumDOutMax=[]  DifferentiatorOutMin=[]  DifferentiatorOutMax=[]  FilterDiffOutCoefMin=[]  FilterDiffOutCoefMax=[]  ReciprocalOutMin=[]  ReciprocalOutMax=[]  SumDenOutMin=[]  SumDenOutMax=[]  SumNumOutMin=[]  SumNumOutMax=[]  DivideOutMin=[]  DivideOutMax=[]  UdiffTsProdOutMin=[]  UdiffTsProdOutMax=[]  NTsProdOutMin=[]  NTsProdOutMax=[]  UintegralTsProdOutMin=[]  UintegralTsProdOutMax=[]  UngainTsProdOutMin=[]  UngainTsProdOutMax=[]  ClampingZeroOutDataTypeStr=Inherit: Inherit via back propagation  ClampingZeroOutMin=[]  ClampingZeroOutMax=[]  FilterDenConstantOutDataTypeStr=Inherit: Inherit via back propagation  FilterDenConstantOutMin=[]  FilterDenConstantOutMax=[]  PCopyOutDataTypeStr=Inherit: Inherit via back propagation  PCopyOutMin=[]  PCopyOutMax=[]  NCopyOutDataTypeStr=Inherit: Inherit via back propagation  NCopyOutMin=[]  NCopyOutMax=[]  IntegratorContinuousStateAttributes=''  IntegratorStateMustResolveToSignalObject=off  IntegratorRTWStateStorageClass=Auto  FilterContinuousStateAttributes=''  FilterStateMustResolveToSignalObject=off  FilterRTWStateStorageClass=Auto  ParallelPVariant=InternalParameters  IdealPVariant=Disabled  IVariant=InternalParameters  DVariant=InternalParameters  IntegratorVariant=Continuous  SatVariant=Disabled  AWVariant=Passthrough  PCopyVariant=Disabled  TRVariant=Disabled  FdbkBlocksVariant=Forward  IdealPFdbkVariant=Disabled  SatFdbkVariant=Disabled  DerivativeFilterVariant=ContFilter  NVariant=InternalParameters  NCopyVariant=Disabled  FilterICVariant=InternalICsFilter  IntegratorICVariant=InternalICs  ExternalResetVariant=Disabled  TRSumVariant=Passthrough  SumFdbkVariant=Disabled  SumVariant=Sum_PID  TsampFilterVariant=InternalTs  TsampNgainVariant=Passthrough  TsampIntegralVariant=Disabled_SignalSpec  ExternalSaturationOutDataTypeStr=Inherit: Same as second input  DerivativeSourceVariant=ErrorSignal  PreIntVariant=InternalPreInt
  PID_w : slpidlib/PID Controller  Controller=PID  Form=Parallel  TimeDomain=Continuous-time  UseExternalTs=off  SampleTime=-1  IntegratorMethod=Forward Euler  FilterMethod=Forward Euler  ControllerParametersSource=internal  P=Kp_w  I=Ki_w  UseKiTs=off  D=0  UseExternalDerivativeSource=off  N=100  UseFilter=on  TunerSelectOption=Transfer Function Based (PID Tuner App)  InitialConditionSource=internal  InitialConditionForIntegrator=0  InitialConditionForFilter=0  DifferentiatorICPrevScaledInput=0  ExternalReset=none  TrackingMode=off  Kt=1  LimitOutput=off  SatLimitsSource=internal  UpperSaturationLimit=inf  LowerSaturationLimit=-inf  LinearizeAsGain=on  AntiWindupMode=none  Kb=1  LimitIntegrator=off  UpperIntegratorSaturationLimit=inf  LowerIntegratorSaturationLimit=-inf  POutMin=[]  POutMax=[]  IOutMin=[]  IOutMax=[]  DOutMin=[]  DOutMax=[]  NOutMin=[]  NOutMax=[]  SumOutMin=[]  SumOutMax=[]  SaturationOutMin=[]  SaturationOutMax=[]  PParamMin=[]  PParamMax=[]  IParamMin=[]  IParamMax=[]  DParamMin=[]  DParamMax=[]  NParamMin=[]  NParamMax=[]  KbParamMin=[]  KbParamMax=[]  KtParamMin=[]  KtParamMax=[]  KbOutMin=[]  KbOutMax=[]  KtOutMin=[]  KtOutMax=[]  IntegratorOutMin=[]  IntegratorOutMax=[]  FilterOutMin=[]  FilterOutMax=[]  SumI1OutMin=[]  SumI1OutMax=[]  SumI2OutMin=[]  SumI2OutMax=[]  SumI3OutMin=[]  SumI3OutMax=[]  SumI4OutMin=[]  SumI4OutMax=[]  SumDOutMin=[]  SumDOutMax=[]  DifferentiatorOutMin=[]  DifferentiatorOutMax=[]  FilterDiffOutCoefMin=[]  FilterDiffOutCoefMax=[]  ReciprocalOutMin=[]  ReciprocalOutMax=[]  SumDenOutMin=[]  SumDenOutMax=[]  SumNumOutMin=[]  SumNumOutMax=[]  DivideOutMin=[]  DivideOutMax=[]  UdiffTsProdOutMin=[]  UdiffTsProdOutMax=[]  NTsProdOutMin=[]  NTsProdOutMax=[]  UintegralTsProdOutMin=[]  UintegralTsProdOutMax=[]  UngainTsProdOutMin=[]  UngainTsProdOutMax=[]  ClampingZeroOutDataTypeStr=Inherit: Inherit via back propagation  ClampingZeroOutMin=[]  ClampingZeroOutMax=[]  FilterDenConstantOutDataTypeStr=Inherit: Inherit via back propagation  FilterDenConstantOutMin=[]  FilterDenConstantOutMax=[]  PCopyOutDataTypeStr=Inherit: Inherit via back propagation  PCopyOutMin=[]  PCopyOutMax=[]  NCopyOutDataTypeStr=Inherit: Inherit via back propagation  NCopyOutMin=[]  NCopyOutMax=[]  IntegratorContinuousStateAttributes=''  IntegratorStateMustResolveToSignalObject=off  IntegratorRTWStateStorageClass=Auto  FilterContinuousStateAttributes=''  FilterStateMustResolveToSignalObject=off  FilterRTWStateStorageClass=Auto  ParallelPVariant=InternalParameters  IdealPVariant=Disabled  IVariant=InternalParameters  DVariant=InternalParameters  IntegratorVariant=Continuous  SatVariant=Disabled  AWVariant=Passthrough  PCopyVariant=Disabled  TRVariant=Disabled  FdbkBlocksVariant=Forward  IdealPFdbkVariant=Disabled  SatFdbkVariant=Disabled  DerivativeFilterVariant=ContFilter  NVariant=InternalParameters  NCopyVariant=Disabled  FilterICVariant=InternalICsFilter  IntegratorICVariant=InternalICs  ExternalResetVariant=Disabled  TRSumVariant=Passthrough  SumFdbkVariant=Disabled  SumVariant=Sum_PID  TsampFilterVariant=InternalTs  TsampNgainVariant=Passthrough  TsampIntegralVariant=Disabled_SignalSpec  ExternalSaturationOutDataTypeStr=Inherit: Same as second input  DerivativeSourceVariant=ErrorSignal  PreIntVariant=InternalPreInt
  Sat_Fl : Saturate  UpperLimit=F_max  LowerLimit=-(F_max)
  Sat_Fr : Saturate  UpperLimit=F_max  LowerLimit=-(F_max)
  SpeedErr : MATLAB Function  TreatAsAtomicUnit=on
  TagPoint : MATLAB Function  TreatAsAtomicUnit=on
  TrackLag : StateSpace  A=trk_A  B=trk_B  C=trk_C  D=trk_D  InitialCondition=[0;0]
  compute_u : MATLAB Function  TreatAsAtomicUnit=on
  q_true : Outport
  V_true : Outport  Port=2
  tag scope: V_true=global, q_true=global
  wires:
  C_pwm_dz/1 -> EscInv/2(pwm_dz)
  C_k_pwm/1 -> EscInv/3(k_pwm)
  C_B_eff/1 -> SpeedErr/3(B_eff)
  C_L_r/1 -> SpeedErr/4(L_r)
  C_b_trk/1 -> Control_allocation/3(b_trk)
  C_L_r_2/1 -> Control_allocation/4(L_r)
  Control_allocation/1(Fr) -> Sat_Fr/1
  Control_allocation/2(Fl) -> Sat_Fl/1
  C_alpha_s/1 -> compute_u/2(alpha_s)
  C_dyn_p/1 -> Dynamics/7(dyn_p)
  Clock/1 -> Kinematics/4(t)
  C_dist_p/1 -> Kinematics/5(dist_p)
  C_r_tag/1 -> TagPoint/2(r_tag)
  Sat_Fl/1 -> Dynamics/6(Fl)
  Sat_Fr/1 -> Dynamics/5(Fr)
  Integ_V/1 -> SpeedErr/2(V_act), compute_u/1(V_act), Dynamics/2(V_act), V_true/1, Kinematics/1(V_act), [V_true]
  Dynamics/1(V_dot) -> Integ_V/1
  SpeedErr/2(e_Lw) -> PID_w/1
  SpeedErr/1(e_v) -> PID_v/1
  motor_pwm_rx/1 -> EscInv/1(motor_pwm)
  Integ_q/1 -> Dynamics/1(q), Kinematics/2(q), TagPoint/1(q_c)
  Kinematics/1(q_dot) -> Integ_q/1
  TagPoint/1(q_tag) -> q_true/1, [q_true]
  PID_w/1 -> Control_allocation/2(tau_N)
  PID_v/1 -> Control_allocation/1(tau_X)
  compute_u/1(u) -> Derivative_u/1, Dynamics/3(u), Kinematics/3(u)
  Derivative_u/1 -> Dynamics/4(u_dot)
  TrackLag/1 -> SpeedErr/1(v_trk)
  EscInv/1(v_trk_cmd) -> TrackLag/1

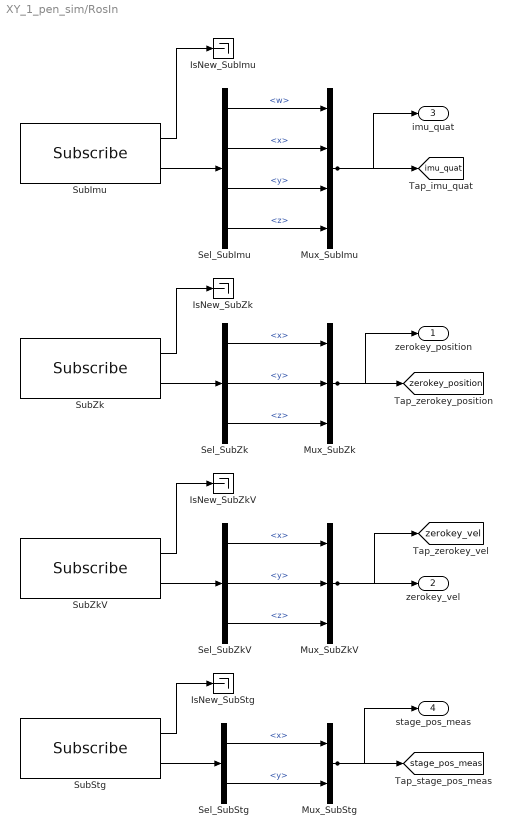
== system XY_1_pen_sim/RosIn ==
  IsNew_SubImu : Terminator
  IsNew_SubStg : Terminator
  IsNew_SubZk : Terminator
  IsNew_SubZkV : Terminator
  Mux_SubImu : Mux
  Mux_SubStg : Mux  Inputs=2
  Mux_SubZk : Mux  Inputs=3
  Mux_SubZkV : Mux  Inputs=3
  Sel_SubImu : BusSelector  OutputSignals=orientation.w,orientation.x,orientation.y,orientation.z
  Sel_SubStg : BusSelector  OutputSignals=point.x,point.y
  Sel_SubZk : BusSelector  OutputSignals=point.x,point.y,point.z
  Sel_SubZkV : BusSelector  OutputSignals=twist.linear.x,twist.linear.y,twist.linear.z
  SubImu : ros2lib/Subscribe  Description=이산: ROS Subscribe 는 구독 주기로만 돈다 / Discrete: ROS Subscribe runs only at the subscription period  topicSource=Specify your own  topic=/imu/data  messageType=sensor_msgs/Imu  sampleTime=Ts_ctrl  QOSHistory=Keep last  QOSDepth=1  QOSReliability=Reliable  QOSDurability=Volatile  QOSDeadline=Inf  QOSLifespan=Inf  QOSLiveliness=Automatic  QOSLeaseDuration=Inf  QOSAvoidROSNamespaceConventions=off
  SubStg : ros2lib/Subscribe  Description=이산: ROS Subscribe 는 구독 주기로만 돈다 / Discrete: ROS Subscribe runs only at the subscription period  topicSource=Specify your own  topic=/stage/pos  messageType=geometry_msgs/PointStamped  sampleTime=Ts_ctrl  QOSHistory=Keep last  QOSDepth=1  QOSReliability=Reliable  QOSDurability=Volatile  QOSDeadline=Inf  QOSLifespan=Inf  QOSLiveliness=Automatic  QOSLeaseDuration=Inf  QOSAvoidROSNamespaceConventions=off
  SubZk : ros2lib/Subscribe  Description=이산: ROS Subscribe 는 구독 주기로만 돈다 / Discrete: ROS Subscribe runs only at the subscription period  topicSource=Specify your own  topic=/zerokey/position  messageType=geometry_msgs/PointStamped  sampleTime=Ts_ctrl  QOSHistory=Keep last  QOSDepth=1  QOSReliability=Reliable  QOSDurability=Volatile  QOSDeadline=Inf  QOSLifespan=Inf  QOSLiveliness=Automatic  QOSLeaseDuration=Inf  QOSAvoidROSNamespaceConventions=off
  SubZkV : ros2lib/Subscribe  Description=이산: ROS Subscribe 는 구독 주기로만 돈다 / Discrete: ROS Subscribe runs only at the subscription period  topicSource=Specify your own  topic=/zerokey/vel  messageType=geometry_msgs/TwistStamped  sampleTime=Ts_ctrl  QOSHistory=Keep last  QOSDepth=1  QOSReliability=Reliable  QOSDurability=Volatile  QOSDeadline=Inf  QOSLifespan=Inf  QOSLiveliness=Automatic  QOSLeaseDuration=Inf  QOSAvoidROSNamespaceConventions=off
  zerokey_position : Outport
  zerokey_vel : Outport  Port=2
  imu_quat : Outport  Port=3
  stage_pos_meas : Outport  Port=4
  tag scope: imu_quat=global, stage_pos_meas=global, zerokey_position=global, zerokey_vel=global
  wires:
  SubZkV/1 -> IsNew_SubZkV/1
  SubZkV/2 -> Sel_SubZkV/1
  SubImu/1 -> IsNew_SubImu/1
  SubImu/2 -> Sel_SubImu/1
  SubZk/1 -> IsNew_SubZk/1
  SubZk/2 -> Sel_SubZk/1
  SubStg/1 -> IsNew_SubStg/1
  SubStg/2 -> Sel_SubStg/1
  Sel_SubImu/1 -> Mux_SubImu/1  "<w>"
  Sel_SubImu/2 -> Mux_SubImu/2  "<x>"
  Sel_SubImu/3 -> Mux_SubImu/3  "<y>"
  Sel_SubImu/4 -> Mux_SubImu/4  "<z>"
  Sel_SubZk/1 -> Mux_SubZk/1  "<x>"
  Sel_SubZk/2 -> Mux_SubZk/2  "<y>"
  Sel_SubZk/3 -> Mux_SubZk/3  "<z>"
  Sel_SubZkV/1 -> Mux_SubZkV/1  "<x>"
  Sel_SubZkV/2 -> Mux_SubZkV/2  "<y>"
  Sel_SubZkV/3 -> Mux_SubZkV/3  "<z>"
  Sel_SubStg/1 -> Mux_SubStg/1  "<x>"
  Sel_SubStg/2 -> Mux_SubStg/2  "<y>"
  Mux_SubImu/1 -> imu_quat/1, [imu_quat]
  Mux_SubZk/1 -> zerokey_position/1, [zerokey_position]
  Mux_SubZkV/1 -> zerokey_vel/1, [zerokey_vel]
  Mux_SubStg/1 -> stage_pos_meas/1, [stage_pos_meas]

== system XY_1_pen_sim/RosOut ==
  motor_pwm : Inport
  stage_target_pos : Inport  Port=2
  Asg_PubPwm : BusAssignment  AssignedSignals=x,y
  Asg_PubStg : BusAssignment  AssignedSignals=x,y
  Blank_PubPwm : ros2lib/Blank Message  messageClass=Message  entityType=geometry_msgs/Point  messageType=geometry_msgs/Point  SampleTime=inf
  Blank_PubStg : ros2lib/Blank Message  messageClass=Message  entityType=geometry_msgs/Point  messageType=geometry_msgs/Point  SampleTime=inf
  Dmx_PubPwm : Demux  Outputs=2
  Dmx_PubStg : Demux  Outputs=2
  PubPwm : ros2lib/Publish  topicSource=Specify your own  topic=/motor_pwm  messageType=geometry_msgs/Point  QOSHistory=Keep last  QOSDepth=1  QOSReliability=Reliable  QOSDurability=Volatile  QOSDeadline=Inf  QOSLifespan=Inf  QOSLiveliness=Automatic  QOSLeaseDuration=Inf  QOSAvoidROSNamespaceConventions=off
  PubStg : ros2lib/Publish  topicSource=Specify your own  topic=/stage/target_pos  messageType=geometry_msgs/Point  QOSHistory=Keep last  QOSDepth=1  QOSReliability=Reliable  QOSDurability=Volatile  QOSDeadline=Inf  QOSLifespan=Inf  QOSLiveliness=Automatic  QOSLeaseDuration=Inf  QOSAvoidROSNamespaceConventions=off
  wires:
  motor_pwm/1 -> Dmx_PubPwm/1
  Dmx_PubStg/2 -> Asg_PubStg/3
  Blank_PubStg/1 -> Asg_PubStg/1
  stage_target_pos/1 -> Dmx_PubStg/1
  Dmx_PubStg/1 -> Asg_PubStg/2
  Blank_PubPwm/1 -> Asg_PubPwm/1
  Dmx_PubPwm/1 -> Asg_PubPwm/2
  Dmx_PubPwm/2 -> Asg_PubPwm/3
  Asg_PubPwm/1 -> PubPwm/1
  Asg_PubStg/1 -> PubStg/1

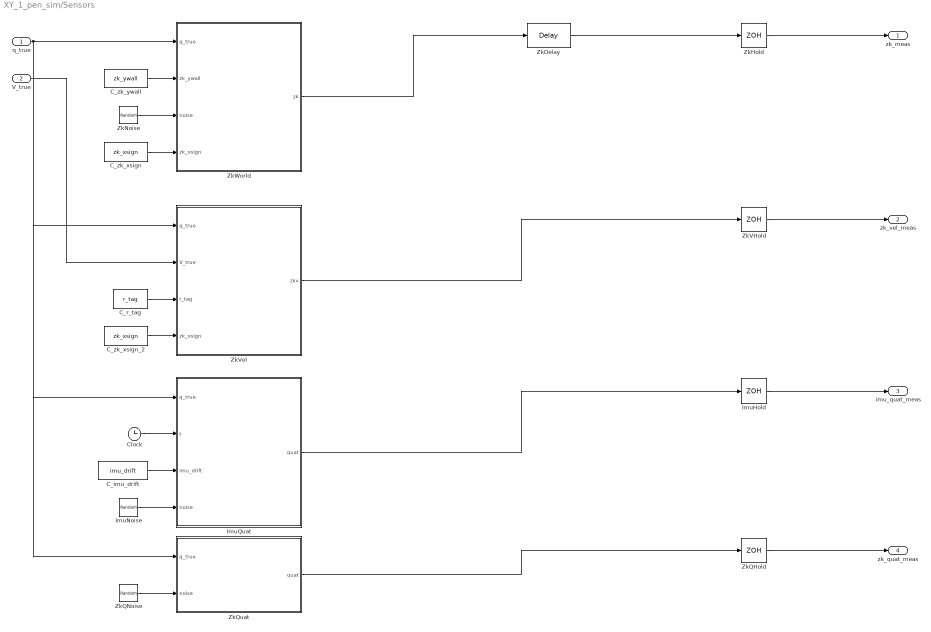
== system XY_1_pen_sim/Sensors ==
  q_true : Inport
  V_true : Inport  Port=2
  C_imu_drift : Constant  Value=imu_drift
  C_r_tag : Constant  Value=r_tag
  C_zk_xsign : Constant  Value=zk_xsign
  C_zk_xsign_2 : Constant  Value=zk_xsign
  C_zk_ywall : Constant  Value=zk_ywall
  Clock : Clock
  ImuHold : ZeroOrderHold  Description=이산: 센서 갱신 주기 (ROS 발행 주기) / Discrete: sensor update period (ROS publish period)  SampleTime=imu_Ts
  ImuNoise : RandomNumber  Description=이산: 센서 잡음은 센서 갱신 주기로 바뀐다 / Discrete: sensor noise changes at the sensor update period  Variance=imu_sigma^2  Seed=21  SampleTime=imu_Ts
  ImuQuat : MATLAB Function  TreatAsAtomicUnit=on
  ZkDelay : TransportDelay  DelayTime=zk_delay  InitialOutput=[zk_xsign*q0(1); zk_ywall; q0(2)]
  ZkHold : ZeroOrderHold  Description=이산: 센서 갱신 주기 (ROS 발행 주기) / Discrete: sensor update period (ROS publish period)  SampleTime=zk_Ts
  ZkNoise : RandomNumber  Description=이산: 센서 잡음은 센서 갱신 주기로 바뀐다 / Discrete: sensor noise changes at the sensor update period  Variance=zk_sigma^2  Seed=[11 12 13]  SampleTime=zk_Ts
  ZkQHold : ZeroOrderHold  Description=이산: 센서 갱신 주기 (ROS 발행 주기) / Discrete: sensor update period (ROS publish period)  SampleTime=zk_Ts
  ZkQNoise : RandomNumber  Description=이산: 센서 잡음은 센서 갱신 주기로 바뀐다 / Discrete: sensor noise changes at the sensor update period  Variance=(3*imu_sigma)^2  Seed=31  SampleTime=zk_Ts
  ZkQuat : MATLAB Function  TreatAsAtomicUnit=on
  ZkVHold : ZeroOrderHold  Description=이산: 센서 갱신 주기 (ROS 발행 주기) / Discrete: sensor update period (ROS publish period)  SampleTime=zk_Ts
  ZkVel : MATLAB Function  TreatAsAtomicUnit=on
  ZkWorld : MATLAB Function  TreatAsAtomicUnit=on
  zk_meas : Outport
  zk_vel_meas : Outport  Port=2
  imu_quat_meas : Outport  Port=3
  zk_quat_meas : Outport  Port=4
  wires:
  C_zk_ywall/1 -> ZkWorld/2(zk_ywall)
  ZkNoise/1 -> ZkWorld/3(noise)
  C_zk_xsign/1 -> ZkWorld/4(zk_xsign)
  ZkHold/1 -> zk_meas/1
  C_r_tag/1 -> ZkVel/3(r_tag)
  C_zk_xsign_2/1 -> ZkVel/4(zk_xsign)
  ZkVHold/1 -> zk_vel_meas/1
  Clock/1 -> ImuQuat/2(t)
  C_imu_drift/1 -> ImuQuat/3(imu_drift)
  ImuNoise/1 -> ImuQuat/4(noise)
  ImuHold/1 -> imu_quat_meas/1
  ZkQNoise/1 -> ZkQuat/2(noise)
  ZkQHold/1 -> zk_quat_meas/1
  V_true/1 -> ZkVel/2(V_true)
  q_true/1 -> ZkWorld/1(q_true), ZkVel/1(q_true), ImuQuat/1(q_true), ZkQuat/1(q_true)
  ImuQuat/1(quat) -> ImuHold/1
  ZkDelay/1 -> ZkHold/1
  ZkWorld/1(zk) -> ZkDelay/1
  ZkQuat/1(quat) -> ZkQHold/1
  ZkVel/1(zkv) -> ZkVHold/1

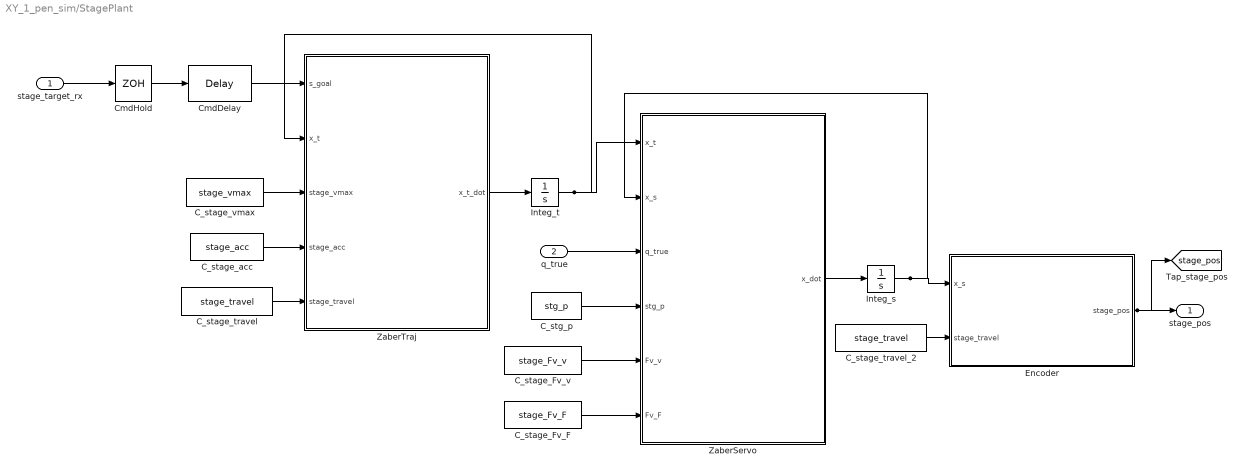
== system XY_1_pen_sim/StagePlant ==
  stage_target_rx : Inport
  q_true : Inport  Port=2
  C_stage_Fv_F : Constant  Value=stage_Fv_F
  C_stage_Fv_v : Constant  Value=stage_Fv_v
  C_stage_acc : Constant  Value=stage_acc
  C_stage_travel : Constant  Value=stage_travel
  C_stage_travel_2 : Constant  Value=stage_travel
  C_stage_vmax : Constant  Value=stage_vmax
  C_stg_p : Constant  Value=stg_p
  CmdDelay : TransportDelay  DelayTime=stage_delay  InitialOutput=[stage_c; stage_c]
  CmdHold : ZeroOrderHold  Description=이산: 스테이지 노드가 move abs 를 보내는 주기 (cmd_rate) / Discrete: period at which the stage node sends move abs (cmd_rate)  SampleTime=stage_cmd_Ts
  Encoder : MATLAB Function  TreatAsAtomicUnit=on
  Integ_s : Integrator  InitialCondition=x_s0
  Integ_t : Integrator  InitialCondition=x_t0
  ZaberServo : MATLAB Function  TreatAsAtomicUnit=on
  ZaberTraj : MATLAB Function  TreatAsAtomicUnit=on
  stage_pos : Outport
  tag scope: stage_pos=global
  wires:
  C_stage_acc/1 -> ZaberTraj/4(stage_acc)
  stage_target_rx/1 -> CmdHold/1
  Integ_t/1 -> ZaberTraj/2(x_t), ZaberServo/1(x_t)
  CmdHold/1 -> CmdDelay/1
  CmdDelay/1 -> ZaberTraj/1(s_goal)
  C_stage_vmax/1 -> ZaberTraj/3(stage_vmax)
  C_stage_travel/1 -> ZaberTraj/5(stage_travel)
  ZaberTraj/1(x_t_dot) -> Integ_t/1
  Integ_s/1 -> ZaberServo/2(x_s), Encoder/1(x_s)
  q_true/1 -> ZaberServo/3(q_true)
  C_stg_p/1 -> ZaberServo/4(stg_p)
  C_stage_Fv_v/1 -> ZaberServo/5(Fv_v)
  C_stage_Fv_F/1 -> ZaberServo/6(Fv_F)
  ZaberServo/1(x_dot) -> Integ_s/1
  C_stage_travel_2/1 -> Encoder/2(stage_travel)
  Encoder/1(stage_pos) -> stage_pos/1, [stage_pos]

== system XY_1_pen_sim/RobotCtrl/M1_GotoStart ==
  WP_target : Inport
  pose : Inport  Port=2
  Enable : EnablePort
  C_K_dist : Constant  Value=K_dist
  C_K_yaw : Constant  Value=K_yaw
  C_r_tag : Constant  Value=r_tag
  Fcn1_GotoStart : MATLAB Function  TreatAsAtomicUnit=on
  Sat_v : Saturate  UpperLimit=v_max  LowerLimit=-(v_max)
  Sat_w : Saturate  UpperLimit=w_max  LowerLimit=-(w_max)
  v : Outport
  w : Outport  Port=2
  wires:
  WP_target/1 -> Fcn1_GotoStart/1(WP_target)
  pose/1 -> Fcn1_GotoStart/2(pose)
  C_K_dist/1 -> Fcn1_GotoStart/3(K_dist)
  C_K_yaw/1 -> Fcn1_GotoStart/4(K_yaw)
  C_r_tag/1 -> Fcn1_GotoStart/5(r_tag)
  Fcn1_GotoStart/1(v) -> Sat_v/1
  Sat_v/1 -> v/1
  Fcn1_GotoStart/2(w) -> Sat_w/1
  Sat_w/1 -> w/1

== system XY_1_pen_sim/RobotCtrl/M2_Turn ==
  WP_prev : Inport
  WP_target : Inport  Port=2
  pose : Inport  Port=3
  Enable : EnablePort
  C_K_yaw : Constant  Value=K_yaw
  Fcn2_Turn : MATLAB Function  TreatAsAtomicUnit=on
  Sat_v : Saturate  UpperLimit=v_max  LowerLimit=-(v_max)
  Sat_w : Saturate  UpperLimit=w_max  LowerLimit=-(w_max)
  v : Outport
  w : Outport  Port=2
  wires:
  WP_prev/1 -> Fcn2_Turn/1(WP_prev)
  WP_target/1 -> Fcn2_Turn/2(WP_target)
  pose/1 -> Fcn2_Turn/3(pose)
  C_K_yaw/1 -> Fcn2_Turn/4(K_yaw)
  Fcn2_Turn/1(v) -> Sat_v/1
  Sat_v/1 -> v/1
  Fcn2_Turn/2(w) -> Sat_w/1
  Sat_w/1 -> w/1

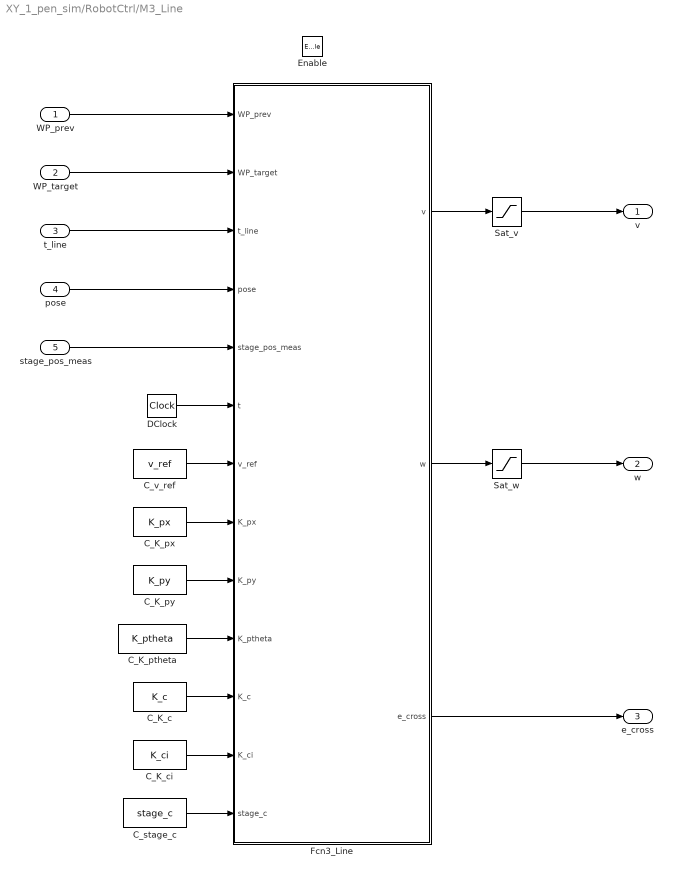
== system XY_1_pen_sim/RobotCtrl/M3_Line ==
  WP_prev : Inport
  WP_target : Inport  Port=2
  t_line : Inport  Port=3
  pose : Inport  Port=4
  stage_pos_meas : Inport  Port=5
  Enable : EnablePort
  C_K_c : Constant  Value=K_c
  C_K_ci : Constant  Value=K_ci
  C_K_ptheta : Constant  Value=K_ptheta
  C_K_px : Constant  Value=K_px
  C_K_py : Constant  Value=K_py
  C_stage_c : Constant  Value=stage_c
  C_v_ref : Constant  Value=v_ref
  DClock : DigitalClock  Description=이산: 제어기 주기의 시간 (Merge 앞 모드 상자 샘플 시간 통일) / Discrete: time at the controller period (common sample time for the mode boxes before Merge)  SampleTime=Ts_ctrl
  Fcn3_Line : MATLAB Function  TreatAsAtomicUnit=on
  Sat_v : Saturate  UpperLimit=v_max  LowerLimit=-(v_max)
  Sat_w : Saturate  UpperLimit=w_max  LowerLimit=-(w_max)
  v : Outport
  w : Outport  Port=2
  e_cross : Outport  Port=3
  wires:
  WP_prev/1 -> Fcn3_Line/1(WP_prev)
  WP_target/1 -> Fcn3_Line/2(WP_target)
  t_line/1 -> Fcn3_Line/3(t_line)
  pose/1 -> Fcn3_Line/4(pose)
  stage_pos_meas/1 -> Fcn3_Line/5(stage_pos_meas)
  DClock/1 -> Fcn3_Line/6(t)
  C_v_ref/1 -> Fcn3_Line/7(v_ref)
  C_K_px/1 -> Fcn3_Line/8(K_px)
  C_K_py/1 -> Fcn3_Line/9(K_py)
  C_K_ptheta/1 -> Fcn3_Line/10(K_ptheta)
  C_K_c/1 -> Fcn3_Line/11(K_c)
  C_K_ci/1 -> Fcn3_Line/12(K_ci)
  C_stage_c/1 -> Fcn3_Line/13(stage_c)
  Fcn3_Line/1(v) -> Sat_v/1
  Sat_v/1 -> v/1
  Fcn3_Line/2(w) -> Sat_w/1
  Sat_w/1 -> w/1
  Fcn3_Line/3(e_cross) -> e_cross/1

== system XY_1_pen_sim/RobotCtrl/M4_Stop ==
  WP_target : Inport
  pose : Inport  Port=2
  Enable : EnablePort
  C_K_dist : Constant  Value=K_dist
  C_K_yaw : Constant  Value=K_yaw
  Fcn4_Stop : MATLAB Function  TreatAsAtomicUnit=on
  Sat_v : Saturate  UpperLimit=v_max  LowerLimit=-(v_max)
  Sat_w : Saturate  UpperLimit=w_max  LowerLimit=-(w_max)
  v : Outport
  w : Outport  Port=2
  wires:
  WP_target/1 -> Fcn4_Stop/1(WP_target)
  pose/1 -> Fcn4_Stop/2(pose)
  C_K_dist/1 -> Fcn4_Stop/3(K_dist)
  C_K_yaw/1 -> Fcn4_Stop/4(K_yaw)
  Fcn4_Stop/1(v) -> Sat_v/1
  Sat_v/1 -> v/1
  Fcn4_Stop/2(w) -> Sat_w/1
  Sat_w/1 -> w/1

== matlab function XY_1_pen_sim/RobotCtrl/M3_Line/Fcn3_Line ==
  data: WP_prev input; v output; WP_target input; t_line input; pose input; stage_pos_meas input; t input; v_ref input; K_px input; K_py input; K_ptheta input; K_c input; K_ci input; stage_c input; w output; e_cross output
function [v, w, e_cross] = Line_Tracking_Mode(WP_prev, WP_target, t_line, pose, stage_pos_meas, t, v_ref, K_px, K_py, K_ptheta, K_c, K_ci, stage_c)
% 모드 3 : 6WP_sim Line_Tracking_Mode — 시간에 따라 앞서 가는 기준점 + 바디 좌표 오차 (게인은 실기 ZeroKey 모델 값)
% Mode 3 : 6WP_sim Line_Tracking_Mode — time-parameterised reference point + body-frame error (real ZeroKey model gains)
% 입력 / Inputs
%   WP_prev, WP_target [2x1, m]  태그 선분 rA -> rB / tag segment
%   t_line [s]  모드 3 진입 시각 / time mode 3 started;   t [s] 현재 시각 / current time
%   pose   [3x1: m, m, rad]  측정 태그 자세 / measured tag pose
%   stage_pos_meas [2x1, mm] /stage/pos (K_c = K_ci = 0 이면 쓰지 않음 / unused when K_c = K_ci = 0)
%   v_ref [m/s] 직선 속도 / line speed;  K_px [1/s];  K_py [rad/(m s)];  K_ptheta [1/s]
%   K_c [-] 스테이지 중앙 유지 비례 / stage-centring P;  K_ci [1/s] 그 적분 / its integral;  stage_c [mm] 스테이지 중앙 / stage centre
% 출력 / Outputs
%   v [m/s], w [rad/s]  속도 명령 / speed commands;   e_cross [m]  바디 좌표 횡오차 e_y / body-frame cross error
% 원리 / Principle
%   x_r = rA + v_ref (t - t_line) u,  [e_x; e_y] = R(psi)^T (x_r - p),  e_th = theta_l - psi
%   v = v_ref cos e_th + K_px e_x,  w = K_py e_y + K_ptheta sin e_th
%   로봇은 옆으로 못 가므로 횡오차 e_y 는 회전(w)으로만 줄인다 / a tracked robot cannot slide sideways, so e_y is removed by turning
th_final = atan2(WP_target(2) - WP_prev(2), WP_target(1) - WP_prev(1));
dist_total = hypot(WP_target(1) - WP_prev(1), WP_target(2) - WP_prev(2));
d_traj = min(v_ref * (t - t_line), dist_total);
x_r = WP_prev(1) + d_traj * cos(th_final);
y_r = WP_prev(2) + d_traj * sin(th_final);
if d_traj < dist_total, vr = v_ref; else, vr = 0; end
theta = pose(3);
err_g = [x_r - pose(1); y_r - pose(2); th_final - theta];
R_mat = [cos(theta) sin(theta) 0; -sin(theta) cos(theta) 0; 0 0 1];
ep = R_mat * err_g;
eth = atan2(sin(ep(3)), cos(ep(3)));
e_cross = ep(2);
v = vr * cos(eth) + K_px * ep(1);
% 스테이지 중앙 유지 (K_c = 0 이면 끔): 스테이지 Y 가 중앙에서 벗어난 만큼을 횡오차에 더해
% 로봇이 펜 쪽으로 다가가게 한다 -> 스테이지가 행정 가운데에서 일한다
% Stage centring (off when K_c = 0): the stage Y offset from centre is added to the cross error
% so the robot moves toward the pen -> the stage works in the middle of its travel
%   비례(K_c) + 적분(K_ci): 적분이 벽면 미끄러짐으로 생기는 정상 편차를 없앤다
%   P (K_c) + I (K_ci): the integral removes the steady offset caused by slip on the wall
persistent I t_prev
if isempty(I), I = 0; t_prev = t; end
e_s = (stage_pos_meas(2) - stage_c) / 1000;   % 스테이지 Y 편차 [m] / stage Y offset [m]
I = I + K_ci * e_s * max(t - t_prev, 0);  t_prev = t;
e_c = ep(2) + K_c * e_s + I;
w = K_py * e_c + K_ptheta * sin(eth);

== matlab function XY_1_pen_sim/RobotCtrl/M4_Stop/Fcn4_Stop ==
  data: WP_target input; v output; pose input; K_dist input; K_yaw input; w output
function [v, w] = Stop_Destination_Mode(WP_target, pose, K_dist, K_yaw)
% 모드 4 : 6WP_sim Stop_Destination_Mode — 끝점(WP_target) 으로 Goto 식을 계속 돌려 그 자리에 머문다
% Mode 4 : 6WP_sim Stop_Destination_Mode — keeps running the go-to law on the end point to hold position
% 입력 / Inputs : WP_target = rB [2x1, m], pose [m, m, rad], K_dist [1/s], K_yaw [1/s]
% 출력 / Outputs: v [m/s], w [rad/s]  (끝점 10 mm 안에서는 w = 0 / w = 0 within 10 mm of the end point)
err_x = WP_target(1) - pose(1);  err_y = WP_target(2) - pose(2);
dist = hypot(err_x, err_y);
target_th = atan2(err_y, err_x);
a = atan2(sin(target_th - pose(3)), cos(target_th - pose(3)));
v = K_dist * dist * max(0, cos(a));
w = K_yaw * a + 0.5 * sin(a) * cos(a);
if dist < 0.01, w = 0; end                     % 끝점 위에서는 방향을 돌리지 않는다 / no turning on the end point

== matlab function XY_1_pen_sim/PwmMap/calc_pwm ==
  data: v_cmd input; motor_pwm output; w_cmd input; v_full input; w_full input; db_v input; db_w input
function motor_pwm = calc_pwm(v_cmd, w_cmd, v_full, w_full, db_v, db_w)
% calc_pwm : 차체 속도 명령 -> 좌우 모터 PWM (실기 MATLAB Function6 calc_pwm 과 같은 식)
% calc_pwm : body speed command -> left/right motor PWM (same as the real MATLAB Function6 calc_pwm)
% 입력 / Inputs
%   v_cmd  [m/s]    전진 속도 명령 (RobotCtrl) / forward speed command
%   w_cmd  [rad/s]  요 각속도 명령, 반시계 (왼쪽으로 돎) + / yaw-rate command, CCW (turning left) +
%   v_full [m/s]    throttle 400 count 일 때 궤도 속도 (0.20) / track speed at 400 counts of throttle
%   w_full [rad/s]  steer 400 count 일 때 요 각속도 (1.37) / yaw rate at 400 counts of steer
%   db_v, db_w [count]  ESC 데드밴드 역보상 크기 (47, 20) / ESC dead-band pre-compensation
% 출력 / Output
%   motor_pwm [2x1, count]  [왼쪽; 오른쪽] 서보 펄스 폭 [us] 와 같은 수, 1500 = 정지, 1100-1900
%                           [left; right] servo pulse width in microseconds, 1500 = stop, 1100-1900
%                           -> /motor_pwm (geometry_msgs/Point x, y) -> Arduino Mega -> C620 ESC
% 원리 / Principle
%   1) 실기에서는 PID 출력 (-0.5 ~ 0.5, 단위 없음) 이 V, W 로 들어간다. 1 판에는 내부 PID 가 없으므로
%      속도 명령을 같은 범위로 정규화: V = 0.5 v_cmd / v_full
%      The real model feeds PID outputs (-0.5 to 0.5, unitless) as V, W. v1 has no inner PID, so the
%      speed commands are normalised to the same range: V = 0.5 v_cmd / v_full
%   2) throttle = db tanh(V/0.02) + (400 - db) V/0.5 : 0 근처에서 db 만큼 뛰어 ESC 데드존을 건너뛴다
%      throttle jumps by db near zero to step over the ESC dead zone, then rises linearly to 400
%   3) left = throttle - steer, right = throttle + steer (steer > 0 이면 오른쪽이 빨라 왼쪽으로 돈다)
%      (steer > 0: the right track is faster, so the robot turns left)
%   4) 오른쪽 모터는 거울 대칭으로 달려 있어 부호를 뒤집는다 / the right motor is mirrored, so its sign is inverted
V = max(-0.5, min(0.5, 0.5 * v_cmd / v_full));
W = max(-0.5, min(0.5, 0.5 * w_cmd / w_full));
NEUTRAL = 1500;  MAX_OFFSET = 400;  V_EPS = 0.02;  W_EPS = 0.10;
db_v_c = max(0, min(MAX_OFFSET, db_v));
db_w_c = max(0, min(MAX_OFFSET, db_w));
throttle = db_v_c * tanh(V / V_EPS) + (MAX_OFFSET - db_v_c) * (V / 0.5);
steer    = db_w_c * tanh(W / W_EPS) + (MAX_OFFSET - db_w_c) * (W / 0.5);
left_raw  = throttle - steer;
right_raw = throttle + steer;
right_inv = -right_raw;                         % 우측 모터 물리적 반전 / right motor physically inverted
motor_pwm = [max(1100, min(1900, NEUTRAL + left_raw));
             max(1100, min(1900, NEUTRAL + right_inv))];
